simulink model "DeltaRobot_V2"  (R2026a)
settings: Solver=VariableStepAuto  StopTime=circ.Tend  AbsTol=1e-3  EnableMultiTasking=on
PostLoadFcn:
  | mbroot = fileparts(fileparts(get_param(bdroot,'FileName')));
  | addpath(fullfile(mbroot,'model'), fullfile(mbroot,'lib'), mbroot);
InitFcn:
  | mbroot = fileparts(fileparts(get_param(bdroot,'FileName')));
  | addpath(fullfile(mbroot,'model'), fullfile(mbroot,'lib'), mbroot);
  | delta_init(mbroot);
undefined symbols (not defined in the file): circ, geom
libraries: nesl_utility x19, sm_lib x8
settings Model: Creator=bzbos  LastModifiedBy=bzbos
settings DebuggingCC: SubsystemReferenceDiagnosticForUnitTest=warning
settings SimscapeCC: SimscapeNominalValues="[{\"value\":\"1\",\"unit\":\"A\"},{\"value\":\"1\",\"unit\":\"bar\"},{\"value\":\"1\",\"unit\":\"cm^2\"},{\"value\":\"1\",\"unit\":\"cm^3/s\"},{\"value\":\"1\",\"unit\":\"kJ/kg\"},{\"value\":\"1\",\"unit\":\"kW\"},{\"value\":\"1\",\"unit\":\"l\"},{\"value\":\"1\",\"unit\":\"N\"},{\"value\":\"1\",\"unit\":\"N*m\"},{\"value\":\"1\",\"unit\":\"V\"}]"  SimscapeLogType=none

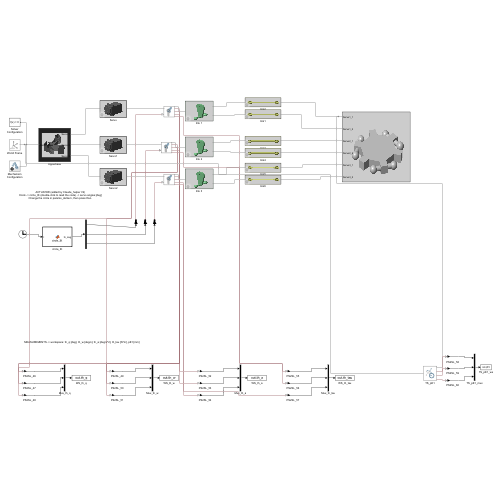
[thumbnail: Simulink's stored preview of the top-level diagram]
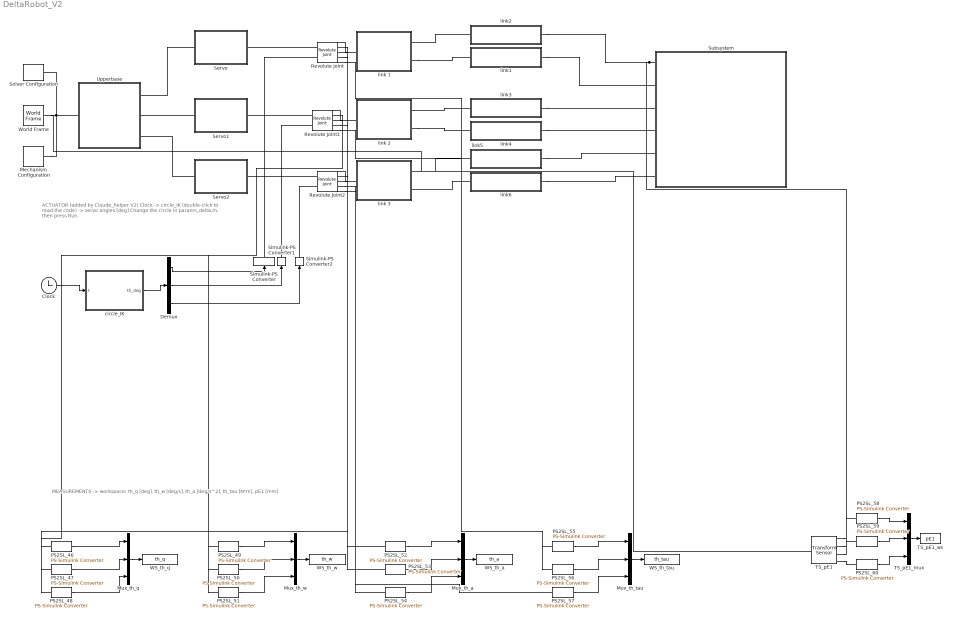
== system DeltaRobot_V2 ==
  note: ACTUATOR (added by Claude_helper V2)
      | Clock -> circle_IK (double-click to read the code) -> servo angles [deg]
      | Change the circle in params_delta.m, then press Run.
  note: MEASUREMENTS -> workspace: th_q [deg], th_w [deg/s], th_a [deg/s^2], th_tau [N*m], pE1 [mm]
  Clock : Clock
  Demux : Demux  Outputs=3
  Mechanism Configuration : sm_lib/Utilities/Mechanism Configuration  UniformGravity=Constant  GravityVector=[0 -9.80665 0 ]  GravityVectorUnits=m/s^2  LinearizationDelta=0.001  JointModeTransitionNonlinearIterations=2
  Mux_th_a : Mux  Inputs=3
  Mux_th_q : Mux  Inputs=3
  Mux_th_tau : Mux  Inputs=3
  Mux_th_w : Mux  Inputs=3
  PS2SL_46 : nesl_utility/PS-Simulink Converter  PhysicalDomain=network_engine_domain  SubClassName=ps_output  LeftPortType=input  RightPortType=output  PseudoPeriodic=off  Frequencies=[]  VectorFormat=inherit  Unit=deg  AffineConversion=off
  PS2SL_47 : nesl_utility/PS-Simulink Converter  PhysicalDomain=network_engine_domain  SubClassName=ps_output  LeftPortType=input  RightPortType=output  PseudoPeriodic=off  Frequencies=[]  VectorFormat=inherit  Unit=deg  AffineConversion=off
  PS2SL_48 : nesl_utility/PS-Simulink Converter  PhysicalDomain=network_engine_domain  SubClassName=ps_output  LeftPortType=input  RightPortType=output  PseudoPeriodic=off  Frequencies=[]  VectorFormat=inherit  Unit=deg  AffineConversion=off
  PS2SL_49 : nesl_utility/PS-Simulink Converter  PhysicalDomain=network_engine_domain  SubClassName=ps_output  LeftPortType=input  RightPortType=output  PseudoPeriodic=off  Frequencies=[]  VectorFormat=inherit  Unit=deg/s  AffineConversion=off
  PS2SL_50 : nesl_utility/PS-Simulink Converter  PhysicalDomain=network_engine_domain  SubClassName=ps_output  LeftPortType=input  RightPortType=output  PseudoPeriodic=off  Frequencies=[]  VectorFormat=inherit  Unit=deg/s  AffineConversion=off
  PS2SL_51 : nesl_utility/PS-Simulink Converter  PhysicalDomain=network_engine_domain  SubClassName=ps_output  LeftPortType=input  RightPortType=output  PseudoPeriodic=off  Frequencies=[]  VectorFormat=inherit  Unit=deg/s  AffineConversion=off
  PS2SL_52 : nesl_utility/PS-Simulink Converter  PhysicalDomain=network_engine_domain  SubClassName=ps_output  LeftPortType=input  RightPortType=output  PseudoPeriodic=off  Frequencies=[]  VectorFormat=inherit  Unit=deg/s^2  AffineConversion=off
  PS2SL_53 : nesl_utility/PS-Simulink Converter  PhysicalDomain=network_engine_domain  SubClassName=ps_output  LeftPortType=input  RightPortType=output  PseudoPeriodic=off  Frequencies=[]  VectorFormat=inherit  Unit=deg/s^2  AffineConversion=off
  PS2SL_54 : nesl_utility/PS-Simulink Converter  PhysicalDomain=network_engine_domain  SubClassName=ps_output  LeftPortType=input  RightPortType=output  PseudoPeriodic=off  Frequencies=[]  VectorFormat=inherit  Unit=deg/s^2  AffineConversion=off
  PS2SL_55 : nesl_utility/PS-Simulink Converter  PhysicalDomain=network_engine_domain  SubClassName=ps_output  LeftPortType=input  RightPortType=output  PseudoPeriodic=off  Frequencies=[]  VectorFormat=inherit  Unit=N*m  AffineConversion=off
  PS2SL_56 : nesl_utility/PS-Simulink Converter  PhysicalDomain=network_engine_domain  SubClassName=ps_output  LeftPortType=input  RightPortType=output  PseudoPeriodic=off  Frequencies=[]  VectorFormat=inherit  Unit=N*m  AffineConversion=off
  PS2SL_57 : nesl_utility/PS-Simulink Converter  PhysicalDomain=network_engine_domain  SubClassName=ps_output  LeftPortType=input  RightPortType=output  PseudoPeriodic=off  Frequencies=[]  VectorFormat=inherit  Unit=N*m  AffineConversion=off
  PS2SL_58 : nesl_utility/PS-Simulink Converter  PhysicalDomain=network_engine_domain  SubClassName=ps_output  LeftPortType=input  RightPortType=output  PseudoPeriodic=off  Frequencies=[]  VectorFormat=inherit  Unit=mm  AffineConversion=off
  PS2SL_59 : nesl_utility/PS-Simulink Converter  PhysicalDomain=network_engine_domain  SubClassName=ps_output  LeftPortType=input  RightPortType=output  PseudoPeriodic=off  Frequencies=[]  VectorFormat=inherit  Unit=mm  AffineConversion=off
  PS2SL_60 : nesl_utility/PS-Simulink Converter  PhysicalDomain=network_engine_domain  SubClassName=ps_output  LeftPortType=input  RightPortType=output  PseudoPeriodic=off  Frequencies=[]  VectorFormat=inherit  Unit=mm  AffineConversion=off
  Revolute Joint : sm_lib/Joints/Revolute Joint  JointMode=Normal  CompositeWrenchDir=FollowerOnBase  CompositeWrenchFrame=BaseFrame  SenseConstraintForce=off  SenseConstraintTorque=off  SenseTotalForce=off  SenseTotalTorque=off  PositionTargetSpecify=off  PositionTargetPriority=High  PositionTargetValue=0  PositionTargetValueUnits=deg  VelocityTargetSpecify=off  VelocityTargetPriority=High  VelocityTargetValue=0  VelocityTargetValueUnits=deg/s  EquilibriumPosition=-40  EquilibriumPositionUnits=deg  SpringStiffness=0  SpringStiffnessUnits=N*m/deg  DampingCoefficient=0  DampingCoefficientUnits=N*m/(deg/s)  LowerLimitSpecify=off  LowerLimitBound=-90  LowerLimitBoundUnits=deg  LowerLimitStiffness=1e4  LowerLimitStiffnessUnits=N*m/deg  LowerLimitDamping=10  LowerLimitDampingUnits=N*m/(deg/s)  LowerLimitTransitionRegionWidth=0.1  LowerLimitTransitionRegionWidthUnits=deg  UpperLimitSpecify=off  UpperLimitBound=90  UpperLimitBoundUnits=deg  UpperLimitStiffness=1e4  UpperLimitStiffnessUnits=N*m/deg  UpperLimitDamping=10  UpperLimitDampingUnits=N*m/(deg/s)  UpperLimitTransitionRegionWidth=0.1  UpperLimitTransitionRegionWidthUnits=deg  TorqueActuationMode=ComputedTorque  MotionActuationMode=InputMotion  SensePosition=on  SenseVelocity=on  SenseAcceleration=on  SenseTorqueForce=on  SenseLowerLimitTorqueForce=off  SenseUpperLimitTorqueForce=off
  Revolute Joint1 : sm_lib/Joints/Revolute Joint  JointMode=Normal  CompositeWrenchDir=FollowerOnBase  CompositeWrenchFrame=BaseFrame  SenseConstraintForce=off  SenseConstraintTorque=off  SenseTotalForce=off  SenseTotalTorque=off  PositionTargetSpecify=off  PositionTargetPriority=High  PositionTargetValue=0  PositionTargetValueUnits=deg  VelocityTargetSpecify=off  VelocityTargetPriority=High  VelocityTargetValue=0  VelocityTargetValueUnits=deg/s  EquilibriumPosition=0  EquilibriumPositionUnits=deg  SpringStiffness=0  SpringStiffnessUnits=N*m/deg  DampingCoefficient=0  DampingCoefficientUnits=N*m/(deg/s)  LowerLimitSpecify=off  LowerLimitBound=-90  LowerLimitBoundUnits=deg  LowerLimitStiffness=1e4  LowerLimitStiffnessUnits=N*m/deg  LowerLimitDamping=10  LowerLimitDampingUnits=N*m/(deg/s)  LowerLimitTransitionRegionWidth=0.1  LowerLimitTransitionRegionWidthUnits=deg  UpperLimitSpecify=off  UpperLimitBound=90  UpperLimitBoundUnits=deg  UpperLimitStiffness=1e4  UpperLimitStiffnessUnits=N*m/deg  UpperLimitDamping=10  UpperLimitDampingUnits=N*m/(deg/s)  UpperLimitTransitionRegionWidth=0.1  UpperLimitTransitionRegionWidthUnits=deg  TorqueActuationMode=ComputedTorque  MotionActuationMode=InputMotion  SensePosition=on  SenseVelocity=on  SenseAcceleration=on  SenseTorqueForce=on  SenseLowerLimitTorqueForce=off  SenseUpperLimitTorqueForce=off
  Revolute Joint2 : sm_lib/Joints/Revolute Joint  JointMode=Normal  CompositeWrenchDir=FollowerOnBase  CompositeWrenchFrame=BaseFrame  SenseConstraintForce=off  SenseConstraintTorque=off  SenseTotalForce=off  SenseTotalTorque=off  PositionTargetSpecify=off  PositionTargetPriority=High  PositionTargetValue=0  PositionTargetValueUnits=deg  VelocityTargetSpecify=off  VelocityTargetPriority=High  VelocityTargetValue=0  VelocityTargetValueUnits=deg/s  EquilibriumPosition=0  EquilibriumPositionUnits=deg  SpringStiffness=0  SpringStiffnessUnits=N*m/deg  DampingCoefficient=0  DampingCoefficientUnits=N*m/(deg/s)  LowerLimitSpecify=off  LowerLimitBound=-90  LowerLimitBoundUnits=deg  LowerLimitStiffness=1e4  LowerLimitStiffnessUnits=N*m/deg  LowerLimitDamping=10  LowerLimitDampingUnits=N*m/(deg/s)  LowerLimitTransitionRegionWidth=0.1  LowerLimitTransitionRegionWidthUnits=deg  UpperLimitSpecify=off  UpperLimitBound=90  UpperLimitBoundUnits=deg  UpperLimitStiffness=1e4  UpperLimitStiffnessUnits=N*m/deg  UpperLimitDamping=10  UpperLimitDampingUnits=N*m/(deg/s)  UpperLimitTransitionRegionWidth=0.1  UpperLimitTransitionRegionWidthUnits=deg  TorqueActuationMode=ComputedTorque  MotionActuationMode=InputMotion  SensePosition=on  SenseVelocity=on  SenseAcceleration=on  SenseTorqueForce=on  SenseLowerLimitTorqueForce=off  SenseUpperLimitTorqueForce=off
  Servo : Subsystem  ReferencedSubsystem=Servo_V2
      settings: PortSchema="{\"entries\":[{\"content\":{\"sides\":[{\"content\":{\"connectorIds\":[\"LConn2\"]},\"type\":\"ConnectorPlacement.EquallySpacedRectSide\",\"uuid\":\"7d2bb9f6-1d9c-4a82-99c9-91e88c23ff1d\"},{\"content\":{\"connectorIds\":[\"LConn1\"],\"side\":\"RIGHT\"},\"type\":\"ConnectorPlacement.EquallySpacedRectSide\",\"uuid\":\"853bf471-cd7a-4c3b-b125-086963caf9dc\"},{\"content\":{\"side\":\"TOP\"},\"type\":\"ConnectorPlacement.EquallySpacedRectSide\",\"uuid\":\"30c82ac8-a478-4ebc-9885-6b5f2244c780\"}]},\"type\":\"ConnectorPlacement.EquallySpacedConnector\",\"uuid\":\"a81f0fdd-5030-4741-8ea0-216e7fa03bb7\"}],\"packageUris\":[\"http://schema.mathworks.com/mf0/Connector/R2020b\"],\"version\":\"1.0\"}"
  Servo1 : Subsystem  ReferencedSubsystem=Servo_V2
      settings: PortSchema="{\"entries\":[{\"content\":{\"sides\":[{\"content\":{\"connectorIds\":[\"LConn2\"]},\"type\":\"ConnectorPlacement.EquallySpacedRectSide\",\"uuid\":\"7d2bb9f6-1d9c-4a82-99c9-91e88c23ff1d\"},{\"content\":{\"connectorIds\":[\"LConn1\"],\"side\":\"RIGHT\"},\"type\":\"ConnectorPlacement.EquallySpacedRectSide\",\"uuid\":\"853bf471-cd7a-4c3b-b125-086963caf9dc\"},{\"content\":{\"side\":\"TOP\"},\"type\":\"ConnectorPlacement.EquallySpacedRectSide\",\"uuid\":\"30c82ac8-a478-4ebc-9885-6b5f2244c780\"}]},\"type\":\"ConnectorPlacement.EquallySpacedConnector\",\"uuid\":\"a81f0fdd-5030-4741-8ea0-216e7fa03bb7\"}],\"packageUris\":[\"http://schema.mathworks.com/mf0/Connector/R2020b\"],\"version\":\"1.0\"}"
  Servo2 : Subsystem  ReferencedSubsystem=Servo_V2
      settings: PortSchema="{\"entries\":[{\"content\":{\"sides\":[{\"content\":{\"connectorIds\":[\"LConn2\"]},\"type\":\"ConnectorPlacement.EquallySpacedRectSide\",\"uuid\":\"7d2bb9f6-1d9c-4a82-99c9-91e88c23ff1d\"},{\"content\":{\"connectorIds\":[\"LConn1\"],\"side\":\"RIGHT\"},\"type\":\"ConnectorPlacement.EquallySpacedRectSide\",\"uuid\":\"853bf471-cd7a-4c3b-b125-086963caf9dc\"},{\"content\":{\"side\":\"TOP\"},\"type\":\"ConnectorPlacement.EquallySpacedRectSide\",\"uuid\":\"30c82ac8-a478-4ebc-9885-6b5f2244c780\"}]},\"type\":\"ConnectorPlacement.EquallySpacedConnector\",\"uuid\":\"a81f0fdd-5030-4741-8ea0-216e7fa03bb7\"}],\"packageUris\":[\"http://schema.mathworks.com/mf0/Connector/R2020b\"],\"version\":\"1.0\"}"
  Simulink-PS Converter : nesl_utility/Simulink-PS Converter  PhysicalDomain=network_engine_domain  SubClassName=ps_input  LeftPortType=input  RightPortType=output  PseudoPeriodic=off  Frequencies=[]  NoiseDistribution=none  NoiseParameters=[]  Unit=deg  AffineConversion=off  FilteringAndDerivatives=filter  SimscapeFilterOrder=2  InputFilterTimeConstant=circ.filterTau  UdotUserProvided=2
  Simulink-PS Converter1 : nesl_utility/Simulink-PS Converter  PhysicalDomain=network_engine_domain  SubClassName=ps_input  LeftPortType=input  RightPortType=output  PseudoPeriodic=off  Frequencies=[]  NoiseDistribution=none  NoiseParameters=[]  Unit=deg  AffineConversion=off  FilteringAndDerivatives=filter  SimscapeFilterOrder=2  InputFilterTimeConstant=circ.filterTau  UdotUserProvided=0
  Simulink-PS Converter2 : nesl_utility/Simulink-PS Converter  PhysicalDomain=network_engine_domain  SubClassName=ps_input  LeftPortType=input  RightPortType=output  PseudoPeriodic=off  Frequencies=[]  NoiseDistribution=none  NoiseParameters=[]  Unit=deg  AffineConversion=off  FilteringAndDerivatives=filter  SimscapeFilterOrder=2  InputFilterTimeConstant=circ.filterTau  UdotUserProvided=0
  Solver Configuration : nesl_utility/Solver Configuration  PhysicalDomain=network_engine_domain  SubClassName=solver  LeftPortType=input  RightPortType=generic  Tones=[]  Harmonics=[]  SimulateNoise=off  Profile=off  UseLocalSampling=off  EnableSwitchedLinearOptims=on  FrequencyDomain=off  UseCCode=off  RelTol=0.001  AbsTol=1e-06  MinStep=1e-09  ToWorkspace=off  RevertToSquareIcSolve=off  NumHomotopyIterations=100  PhasorMode=off  PhasorModeNumHarmonics=1  ConsistencySolver=NEWTON_XTOL_AFTER_FTOL  CanonicalOrdering=UNORDERED  OptimizeIntermediates=UNOPTIMIZED  IndexReductionMethod=DerivativeReplacement  DoDC=off  ResidualTolerance=1e-09  ConsistencyTolSource=GLOBAL  ConsistencyAbsTol=0.001  ConsistencyRelTol=0.001  ConsistencyTolFactor=0.001  UseLocalSolver=off  LocalSolverChoice=NE_BACKWARD_EULER_ADVANCER  ResolveIndetEquations=on  FunctionEvalNumThread=1  LocalSolverSampleTime=0.001  DoFixedCost=off  MaxNonlinIter=3  MaxModeIter=2  ComputeImpulses=off  ImpulseIterations=2  LinearAlgebra=Sparse  LinearAlgebraNumThread=0  EquationFormulation=NE_TIME_EF  DelaysMemoryBudget=1024  AutomaticFiltering=on  FilteringTimeConstant=0.001  PartitionStorageMethod=AS_NEEDED  PartitionMemoryBudget=1024  PartitionMethod=FAST  MultibodyUseLocalSolver=off  MultibodyLocalSolverChoice=ODE1  MultibodyLocalSolverSampleTime=0.001
  Subsystem : Subsystem
      mask Display: image('Picture_Base.png');
  TS_pE1 : sm_lib/Frames and Transforms/Transform Sensor  MeasurementFrame=World  RotationSequence=XYX  SenseAngle=off  SenseAxis=off  SenseQ=off  SenseR=off  SenseRotationSequence=off  SenseOmegaX=off  SenseOmegaY=off  SenseOmegaZ=off  SenseOmega=off  SenseQDot=off  SenseRDot=off  SenseRotationSequenceDot=off  SenseAlphaX=off  SenseAlphaY=off  SenseAlphaZ=off  SenseAlpha=off  SenseQDDot=off  SenseRDDot=off  SenseX=on  SenseY=on  SenseZ=on  SenseXYZ=off  SenseRad=off  SenseAzim=off  SenseDist=off  SenseInc=off  SenseXDot=off  SenseYDot=off  SenseZDot=off  SenseXYZDot=off  SenseRadDot=off  SenseAzimDot=off  SenseDistDot=off  SenseIncDot=off  SenseXDDot=off  SenseYDDot=off  SenseZDDot=off  SenseXYZDDot=off  SenseRadDDot=off  SenseAzimDDot=off  SenseDistDDot=off  SenseIncDDot=off
  TS_pE1_mux : Mux  Inputs=3
  TS_pE1_ws : ToWorkspace  VariableName=pE1  SaveFormat=Timeseries  SampleTime=0.002
  Upperbase : Subsystem
      mask Display: image('Picture_UpperBase.png', [0,0,0,0,80,80]);
  WS_th_a : ToWorkspace  VariableName=th_a  SaveFormat=Timeseries  SampleTime=0.002
  WS_th_q : ToWorkspace  VariableName=th_q  SaveFormat=Timeseries  SampleTime=0.002
  WS_th_tau : ToWorkspace  VariableName=th_tau  SaveFormat=Timeseries  SampleTime=0.002
  WS_th_w : ToWorkspace  VariableName=th_w  SaveFormat=Timeseries  SampleTime=0.002
  World Frame : sm_lib/Frames and Transforms/World Frame
  circle_IK : MATLAB Function  TreatAsAtomicUnit=on
  link 1 : Subsystem  ReferencedSubsystem=link_1_V2
  link 2 : Subsystem  ReferencedSubsystem=link_1_V2
  link 3 : Subsystem  ReferencedSubsystem=link_1_V2
  link{1..6} (6 alike) : Subsystem  ReferencedSubsystem=link2_V2
  wires:
  Clock/1 -> circle_IK/1(t)
  circle_IK/1(th_deg) -> Demux/1
  Demux/1 -> Simulink-PS Converter/1
  Demux/2 -> Simulink-PS Converter1/1
  Demux/3 -> Simulink-PS Converter2/1
  PS2SL_46/1 -> Mux_th_q/1
  PS2SL_47/1 -> Mux_th_q/2
  PS2SL_48/1 -> Mux_th_q/3
  Mux_th_q/1 -> WS_th_q/1
  PS2SL_49/1 -> Mux_th_w/1
  PS2SL_50/1 -> Mux_th_w/2
  PS2SL_51/1 -> Mux_th_w/3
  Mux_th_w/1 -> WS_th_w/1
  PS2SL_52/1 -> Mux_th_a/1
  PS2SL_53/1 -> Mux_th_a/2
  PS2SL_54/1 -> Mux_th_a/3
  Mux_th_a/1 -> WS_th_a/1
  PS2SL_55/1 -> Mux_th_tau/1
  PS2SL_56/1 -> Mux_th_tau/2
  PS2SL_57/1 -> Mux_th_tau/3
  Mux_th_tau/1 -> WS_th_tau/1
  PS2SL_58/1 -> TS_pE1_mux/1
  PS2SL_59/1 -> TS_pE1_mux/2
  PS2SL_60/1 -> TS_pE1_mux/3
  TS_pE1_mux/1 -> TS_pE1_ws/1
  connections:
  World Frame/RConn1 -- TS_pE1/LConn1 -- Upperbase/LConn1 -- Mechanism Configuration/RConn1 -- Solver Configuration/RConn1
  Servo/LConn2 -- Upperbase/RConn1
  Servo1/LConn2 -- Upperbase/RConn2
  Servo2/LConn2 -- Upperbase/RConn3
  Revolute Joint1/LConn1 -- Servo1/LConn1
  Revolute Joint/LConn1 -- Servo/LConn1
  Revolute Joint2/LConn1 -- Servo2/LConn1
  link 1/LConn1 -- Revolute Joint/RConn1
  link 2/LConn1 -- Revolute Joint1/RConn1
  link 3/LConn1 -- Revolute Joint2/RConn1
  link2/LConn1 -- link 1/RConn1
  link 1/RConn2 -- link1/LConn1
  link3/LConn1 -- link 2/RConn1
  link 2/RConn2 -- link4/LConn1
  link5/LConn1 -- link 3/RConn1
  link6/LConn1 -- link 3/RConn2
  Simulink-PS Converter/RConn1 -- Revolute Joint/LConn2
  Simulink-PS Converter1/RConn1 -- Revolute Joint1/LConn2
  Revolute Joint2/LConn2 -- Simulink-PS Converter2/RConn1
  Subsystem/LConn1 -- link2/RConn1 -- TS_pE1/RConn1
  link1/RConn1 -- Subsystem/LConn2
  link3/RConn1 -- Subsystem/LConn3
  link4/RConn1 -- Subsystem/LConn4
  link5/RConn1 -- Subsystem/LConn5
  link6/RConn1 -- Subsystem/LConn6
  Revolute Joint/RConn2 -- PS2SL_46/LConn1
  Revolute Joint1/RConn2 -- PS2SL_47/LConn1
  Revolute Joint2/RConn2 -- PS2SL_48/LConn1
  Revolute Joint/RConn3 -- PS2SL_49/LConn1
  Revolute Joint1/RConn3 -- PS2SL_50/LConn1
  Revolute Joint2/RConn3 -- PS2SL_51/LConn1
  Revolute Joint/RConn4 -- PS2SL_52/LConn1
  Revolute Joint1/RConn4 -- PS2SL_53/LConn1
  Revolute Joint2/RConn4 -- PS2SL_54/LConn1
  Revolute Joint/RConn5 -- PS2SL_55/LConn1
  Revolute Joint1/RConn5 -- PS2SL_56/LConn1
  Revolute Joint2/RConn5 -- PS2SL_57/LConn1
  TS_pE1/RConn2 -- PS2SL_58/LConn1
  TS_pE1/RConn3 -- PS2SL_59/LConn1
  TS_pE1/RConn4 -- PS2SL_60/LConn1

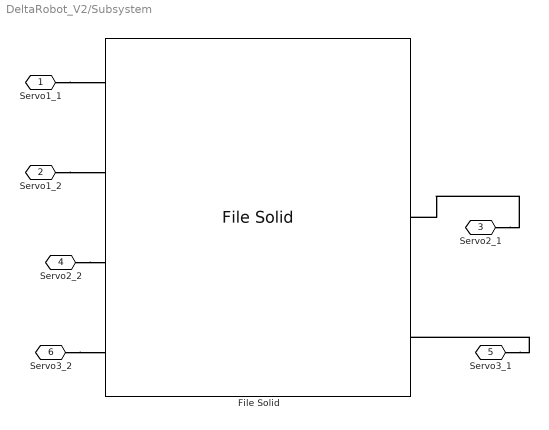
== system DeltaRobot_V2/Subsystem ==
  File Solid : sm_lib/Body Elements/File Solid  ExtGeomFileName=base1.step  UnitType=FromFile  ExtGeomFileUnits=m  StepReaderType=HEX  ExportConvexHullGeometry=off  InertiaType=CalculateFromGeometry  BasedOnType=Mass  Density=1000  DensityUnits=kg/m^3  Mass=30  MassUnits=g  CenterOfMass=[0 0 0]  CenterOfMassUnits=m  MomentsOfInertia=[1 1 1]  MomentsOfInertiaUnits=kg*m^2  ProductsOfInertia=[0 0 0]  ProductsOfInertiaUnits=kg*m^2  GraphicType=FromGeometry  MarkerShape=Sphere  MarkerSize=10  GraphicVisPropType=SimpleVisualProperties  GraphicDiffuseColor=[1 1 1]  GraphicOpacity=1  GraphicSpecularColor=[0.5 0.5 0.5 1.0]  GraphicAmbientColor=[0.15 0.15 0.15 1.0]  GraphicEmissiveColor=[0.0 0.0 0.0 1.0]  GraphicShininess=75  DoExposeReferenceFrame=on  SerializedFrames=|
      | <Frames>
      | 
      |   <Frame>
      |     <Id>Frame1</Id>
      |     <Value>
      |       <Name>Servo1 1</Name>
      |       <Origin>
      |         <Source>GeometricFeature</Source>
      |         <FeatureName>spherical surface 2</FeatureName>
      |       </Origin>
      |       <PrimaryAxis>
      |         <DefinedDirection>-Z</DefinedDirection>
      |         <Source>GeometricFeature</Source>
      |         <SourceDirection>+Z</SourceDirection>
      |         <FeatureName>planar surface 3</FeatureName>
      |       </PrimaryAxis>
      |       <SecondaryAxis>
      |         <DefinedDirection>+X</DefinedDirection>
      |         <Source>GeometricFeature</Source>
      |         <SourceDirection>+X</SourceDirection>
      |         <FeatureName>planar surface 24</FeatureName>
      |       </SecondaryAxis>
      |     </Value>
      |   </Frame>
      | 
      |   <Frame>
      |     <Id>Frame2</Id>
      |     <Value>
      |       <Name>Servo1 2</Name>
      |       <Origin>
      |         <Source>GeometricFeature</Source>
      |         <FeatureName>spherical surface 1</FeatureName>
      |       </Origin>
      |       <PrimaryAxis>
      |         <DefinedDirection>+Z</DefinedDirection>
      |         <Source>GeometricFeature</Source>
      |         <SourceDirection>+Z</SourceDirection>
      |         <FeatureName>planar surface 1</FeatureName>
      |       </PrimaryAxis>
      |       <SecondaryAxis>
      |         <DefinedDirection>+X</DefinedDirection>
      |         <Source>GeometricFeature</Source>
      |         <SourceDirection>+X</SourceDirection>
      |         <FeatureName>planar surface 24</FeatureName>
      |       </SecondaryAxis>
      |     </Value>
      |   </Frame>
      | 
      |   <Frame>
      |     <Id>Frame3</Id>
      |     <Value>
      |       <Name>Servo2 1</Name>
      |       <Origin>
      |         <Source>GeometricFeature</Source>
      |         <FeatureName>spherical surface 4</FeatureName>
      |       </Origin>
      |       <PrimaryAxis>
      |         <DefinedDirection>-Z</DefinedDirection>
      |         <Source>GeometricFeature</Source>
      |         <SourceDirection>+Z</SourceDirection>
      |         <FeatureName>planar surface 18</FeatureName>
      |       </PrimaryAxis>
      |       <SecondaryAxis>
      |         <DefinedDirection>+X</DefinedDirection>
      |         <Source>GeometricFeature</Source>
      |         <SourceDirection>+X</SourceDirection>
      |         <FeatureName>planar surface 24</FeatureName>
      |       </SecondaryAxis>
      |     </Value>
      |   </Frame>
      | 
      |   <Frame>
      |     <Id>Frame4</Id>
      |     <Value>
      |       <Name>Servo2 2</Name>
      |       <Origin>
      |         <Source>GeometricFeature</Source>
      |         <FeatureName>spherical surface 3</FeatureName>
      |       </Origin>
      |       <PrimaryAxis>
      |         <DefinedDirection>-Z</DefinedDirection>
      |         <Source>GeometricFeature</Source>
      |         <SourceDirection>+Z</SourceDirection>
      |         <FeatureName>planar surface 20</FeatureName>
      |       </PrimaryAxis>
      |       <SecondaryAxis>
      |         <DefinedDirection>+X</DefinedDirection>
      |         <Source>GeometricFeature</Source>
      |         <SourceDirection>+X</SourceDirection>
      |         <FeatureName>planar surface 24</FeatureName>
      |       </SecondaryAxis>
      |     </Value>
      |   </Frame>
      | 
      |   <Frame>
      |     <Id>Frame5</Id>
      |     <Value>
      |       <Name>Servo3 1</Name>
      |       <Origin>
      |         <Source>GeometricFeature</Source>
      |         <FeatureName>spherical surface 6</FeatureName>
      |       </Origin>
      |       <PrimaryAxis>
      |         <DefinedDirection>+Z</DefinedDirection>
      |         <Source>GeometricFeature</Source>
      |         <SourceDirection>+Z</SourceDirection>
      |         <FeatureName>planar surface 10</FeatureName>
      |       </PrimaryAxis>
      |       <SecondaryAxis>
      |         <DefinedDirection>+X</DefinedDirection>
      |         <Source>GeometricFeature</Source>
      |         <SourceDirection>+X</SourceDirection>
      |         <FeatureName>planar surface 24</FeatureName>
      |       </SecondaryAxis>
      |     </Value>
      |   </Frame>
      | 
      |   <Frame>
      |     <Id>Frame6</Id>
      |     <Value>
      |       <Name>Servo3 2</Name>
      |       <Origin>
      |         <Source>GeometricFeature</Source>
      |         <FeatureName>spherical surface 5</FeatureName>
      |       </Origin>
      |       <PrimaryAxis>
      |         <DefinedDirection>+Z</DefinedDirection>
      |         <Source>GeometricFeature</Source>
      |         <SourceDirection>+Z</SourceDirection>
      |         <FeatureName>planar surface 12</FeatureName>
      |       </PrimaryAxis>
      |       <SecondaryAxis>
      |         <DefinedDirection>+X</DefinedDirection>
      |         <Source>GeometricFeature</Source>
      |         <SourceDirection>+X</SourceDirection>
      |         <FeatureName>planar surface 24</FeatureName>
      |       </SecondaryAxis>
      |     </Value>
      |   </Frame>
      | 
      | </Frames>
  Servo1_1 : PMIOPort  Side=Left
  Servo1_2 : PMIOPort  Port=2  Side=Left
  Servo2_1 : PMIOPort  Port=3  Side=Left
  Servo2_2 : PMIOPort  Port=4  Side=Left
  Servo3_1 : PMIOPort  Port=5  Side=Left
  Servo3_2 : PMIOPort  Port=6  Side=Left
  connections:
  Servo1_1/RConn1 -- File Solid/LConn1
  Servo2_1/RConn1 -- File Solid/RConn2
  Servo3_1/RConn1 -- File Solid/RConn3
  Servo1_2/RConn1 -- File Solid/LConn2
  Servo2_2/RConn1 -- File Solid/LConn3
  Servo3_2/RConn1 -- File Solid/LConn4

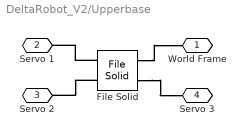
== system DeltaRobot_V2/Upperbase ==
  File Solid : sm_lib/Body Elements/File Solid  ExtGeomFileName=upperbase1.step  UnitType=FromFile  ExtGeomFileUnits=m  StepReaderType=HEX  ExportConvexHullGeometry=off  InertiaType=CalculateFromGeometry  BasedOnType=Mass  Density=1000  DensityUnits=kg/m^3  Mass=60  MassUnits=g  CenterOfMass=[0 0 0]  CenterOfMassUnits=m  MomentsOfInertia=[1 1 1]  MomentsOfInertiaUnits=kg*m^2  ProductsOfInertia=[0 0 0]  ProductsOfInertiaUnits=kg*m^2  GraphicType=FromGeometry  MarkerShape=Sphere  MarkerSize=10  GraphicVisPropType=SimpleVisualProperties  GraphicDiffuseColor=[0.5 0.5 0.5]  GraphicOpacity=1  GraphicSpecularColor=[0.5 0.5 0.5 1.0]  GraphicAmbientColor=[0.15 0.15 0.15 1.0]  GraphicEmissiveColor=[0.0 0.0 0.0 1.0]  GraphicShininess=75  DoExposeReferenceFrame=on  SerializedFrames=|
      | <Frames>
      | 
      |   <Frame>
      |     <Id>Frame1</Id>
      |     <Value>
      |       <Name>F1</Name>
      |       <Origin>
      |         <Source>GeometricFeature</Source>
      |         <FeatureName>circular curve 148</FeatureName>
      |       </Origin>
      |       <PrimaryAxis>
      |         <DefinedDirection>+Z</DefinedDirection>
      |         <Source>GeometricFeature</Source>
      |         <SourceDirection>+Z</SourceDirection>
      |         <FeatureName>circular curve 148</FeatureName>
      |       </PrimaryAxis>
      |       <SecondaryAxis>
      |         <DefinedDirection>+X</DefinedDirection>
      |         <Source>GeometricFeature</Source>
      |         <SourceDirection>+X</SourceDirection>
      |         <FeatureName>planar surface 129</FeatureName>
      |       </SecondaryAxis>
      |     </Value>
      |   </Frame>
      | 
      |   <Frame>
      |     <Id>Frame2</Id>
      |     <Value>
      |       <Name>F2</Name>
      |       <Origin>
      |         <Source>GeometricFeature</Source>
      |         <FeatureName>circular curve 91</FeatureName>
      |       </Origin>
      |       <PrimaryAxis>
      |         <DefinedDirection>+Z</DefinedDirection>
      |         <Source>GeometricFeature</Source>
      |         <SourceDirection>+Z</SourceDirection>
      |         <FeatureName>circular curve 91</FeatureName>
      |       </PrimaryAxis>
      |       <SecondaryAxis>
      |         <DefinedDirection>-X</DefinedDirection>
      |         <Source>GeometricFeature</Source>
      |         <SourceDirection>+X</SourceDirection>
      |         <FeatureName>planar surface 83</FeatureName>
      |       </SecondaryAxis>
      |     </Value>
      |   </Frame>
      | 
      |   <Frame>
      |     <Id>Frame3</Id>
      |     <Value>
      |       <Name>F3</Name>
      |       <Origin>
      |         <Source>GeometricFeature</Source>
      |         <FeatureName>circular curve 205</FeatureName>
      |       </Origin>
      |       <PrimaryAxis>
      |         <DefinedDirection>+Z</DefinedDirection>
      |         <Source>GeometricFeature</Source>
      |         <SourceDirection>+Z</SourceDirection>
      |         <FeatureName>circular curve 205</FeatureName>
      |       </PrimaryAxis>
      |       <SecondaryAxis>
      |         <DefinedDirection>+X</DefinedDirection>
      |         <Source>GeometricFeature</Source>
      |         <SourceDirection>+X</SourceDirection>
      |         <FeatureName>planar surface 36</FeatureName>
      |       </SecondaryAxis>
      |     </Value>
      |   </Frame>
      | 
      | </Frames>
  World Frame : PMIOPort  Side=Left
  Servo 1 : PMIOPort  Port=2  Side=Right
  Servo 2 : PMIOPort  Port=3  Side=Right
  Servo 3 : PMIOPort  Port=4  Side=Right
  connections:
  File Solid/RConn2 -- Servo 3/RConn1
  File Solid/RConn1 -- World Frame/RConn1
  File Solid/LConn2 -- Servo 2/RConn1
  File Solid/LConn1 -- Servo 1/RConn1

== matlab function DeltaRobot_V2/circle_IK ==
  data: t input; th_deg output; circ parameter; geom parameter
function th_deg = circle_IK(t, circ, geom)
% ====================== ACTUATOR OF THE DELTA ROBOT ======================
% Input : t     simulation time [s]
% Param : circ  your variables from params_delta.m
%         geom  robot geometry measured from this model (step1_build_model)
% Output: th_deg  3 servo angles [deg] -> Revolute Joint, Joint1, Joint2
%
% 1) WHERE should the effector be at time t?  (robot frame, mm)
R3 = [geom.ex geom.ey geom.ez];
pHome  = (R3.'*(geom.Xhome - geom.O))*1000;      % home position
pStart = [circ.R; 0; circ.zc];                    % first point on the circle
t1 = circ.Tmove;  t2 = t1 + circ.Tcircle;  t3 = t2 + circ.Tmove;
if t < t1                                         % phase 1: home -> circle
    s = mj(t/circ.Tmove);
    p = pHome + (pStart - pHome)*s;
elseif t < t2                                     % phase 2: circle
    phi = 2*pi*circ.laps*mj((t - t1)/circ.Tcircle);
    p = [circ.R*cos(phi); circ.R*sin(phi); circ.zc];
elseif t < t3                                     % phase 3: circle -> home
    s = mj((t - t2)/circ.Tmove);
    p = pStart + (pHome - pStart)*s;
else                                              % stay at home
    p = pHome;
end
% 2) the same point in the Simscape world frame [m]
X = geom.O + R3*p/1000;
% 3) INVERSE KINEMATICS: which servo angle puts each arm there?
%    rod length must fit:  |X + E_i - C_i(q)| = L2   ->   A cos q + B sin q = K
th_deg = zeros(3,1);
for i = 1:3
    a = geom.a(:,i);  u = geom.u(:,i);  v = cross(a,u);
    D = X + geom.E(:,i) - geom.P(:,i) - geom.d(i)*a;
    A = 2*geom.L1(i)*(u.'*D);
    B = 2*geom.L1(i)*(v.'*D);
    K = D.'*D + geom.L1(i)^2 - geom.L2(i)^2;
    c = min(max(K/sqrt(A^2+B^2), -1), 1);
    q = atan2(B,A) + geom.branch(i)*acos(c);       % elbow-out solution
    qh = geom.qhome(i);
    q = qh + mod(q - qh + pi, 2*pi) - pi;          % keep it near the home angle
    th_deg(i) = q*180/pi;
end
end

function s = mj(x)
% minimum-jerk blend 0 -> 1
x = min(max(x,0),1);
s = 10*x^3 - 15*x^4 + 6*x^5;
end
